simulink model "laba_7_sxema"  (R2025b)
settings: Solver=VariableStepAuto  StartTime=0.0  StopTime=10.0  RelTol=1e-3
settings Model: Creator=user  LastModifiedBy=user

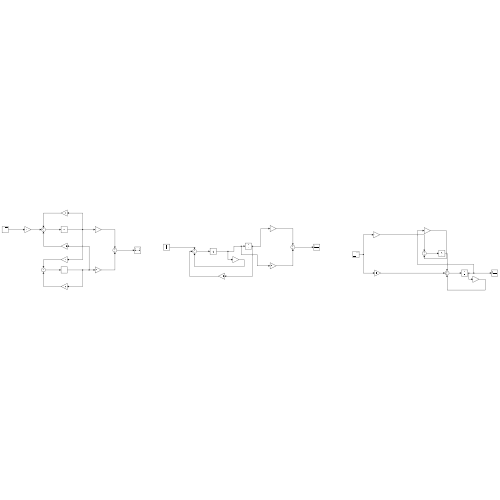
[thumbnail: Simulink's stored preview of the top-level diagram]
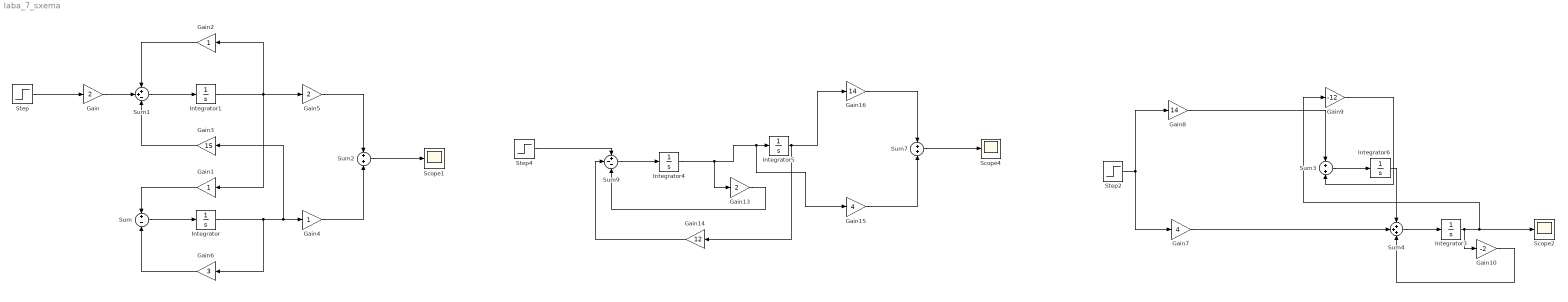
== system laba_7_sxema ==
  Gain : Gain  Gain=2
  Gain1 : Gain
  Gain10 : Gain  Gain=-2
  Gain13 : Gain  Gain=2
  Gain14 : Gain  Gain=12
  Gain15 : Gain  Gain=4
  Gain16 : Gain  Gain=14
  Gain2 : Gain
  Gain3 : Gain  Gain=15
  Gain4 : Gain
  Gain5 : Gain  Gain=2
  Gain6 : Gain  Gain=3
  Gain7 : Gain  Gain=4
  Gain8 : Gain  Gain=14
  Gain9 : Gain  Gain=-12
  Integrator{,1,3..6} (6 alike) : Integrator
  Scope1 : Scope
      settings: ActiveDisplayYMinimum=-0.23000646084626819  ActiveDisplayYMaximum=2.0700581476164142
  Scope2 : Scope
      settings: ActiveDisplayYMinimum=-0.23000646084626819  ActiveDisplayYMaximum=2.0700581476164142  DataLoggingVariableName=ScopeData2
  Scope4 : Scope
      settings: ActiveDisplayYMinimum=-1  ActiveDisplayYMaximum=1  DataLoggingVariableName=ScopeData4
  Step : Step  SampleTime=0
  Step2 : Step  SampleTime=0
  Step4 : Step  SampleTime=0
  Sum : Sum  Inputs=+-
  Sum1 : Sum  Inputs=++-
  Sum2 : Sum
  Sum3 : Sum
  Sum4 : Sum  Inputs=+++
  Sum7 : Sum
  Sum9 : Sum  Inputs=+--
  wires:
  Step/1 -> Gain/1
  Gain/1 -> Sum1/2
  Sum1/1 -> Integrator1/1
  Gain2/1 -> Sum1/1
  Gain3/1 -> Sum1/3
  Integrator1/1 -> Gain1/1, Gain2/1, Gain5/1
  Gain1/1 -> Sum/1
  Gain6/1 -> Sum/2
  Sum/1 -> Integrator/1
  Integrator/1 -> Gain6/1, Gain3/1, Gain4/1
  Sum2/1 -> Scope1/1
  Gain5/1 -> Sum2/1
  Gain4/1 -> Sum2/2
  Gain7/1 -> Sum4/2
  Step2/1 -> Gain8/1, Gain7/1
  Sum4/1 -> Integrator3/1
  Integrator6/1 -> Sum4/1
  Gain9/1 -> Sum3/2
  Sum3/1 -> Integrator6/1
  Integrator3/1 -> Gain9/1, Scope2/1, Gain10/1
  Gain8/1 -> Sum3/1
  Gain10/1 -> Sum4/3
  Sum7/1 -> Scope4/1
  Gain14/1 -> Sum9/2
  Gain13/1 -> Sum9/3
  Sum9/1 -> Integrator4/1
  Integrator5/1 -> Gain16/1, Gain14/1
  Step4/1 -> Sum9/1
  Gain16/1 -> Sum7/1
  Gain15/1 -> Sum7/2
  Integrator4/1 -> Gain15/1, Integrator5/1, Gain13/1
